simulink model "IP_LQR_Design"  (R2025b)
settings: Solver=FixedStepAuto  StartTime=0.0  StopTime=10.0  FixedStep=0.01  RelTol=1e-3
undefined symbols (not defined in the file): b, c, g, I, kb, KK, kt, l, M, m, r, Rm
libraries: vrlib x3
settings Model: Creator=jitendra  LastModifiedBy=joelalfaro
settings SolverCC: AlgebraicLoopSolver=TrustRegion
settings DataIOCC: ExternalInput=getinputstruct(op_trim1)  InitialState=getstatestruct(op_trim1)  ReturnWorkspaceOutputs=off
settings DebuggingCC: UnconnectedInputMsg=warning  UnconnectedOutputMsg=warning  UnconnectedLineMsg=warning  ArithmeticOperatorsInVariantConditions=warning
settings ModelReferenceCC: EnableRefExpFcnMdlSchedulingChecks=on
settings SFSimCC: SimUseLocalCustomCode=off  CustomCodeUndefinedFunction=UseInterfaceOnly
settings RTWCC: RTWUseLocalCustomCode=off  GPUComputeCapability=3.5

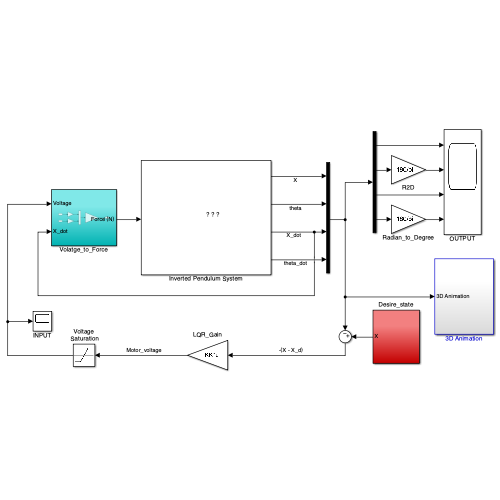
[thumbnail: Simulink's stored preview of the top-level diagram]
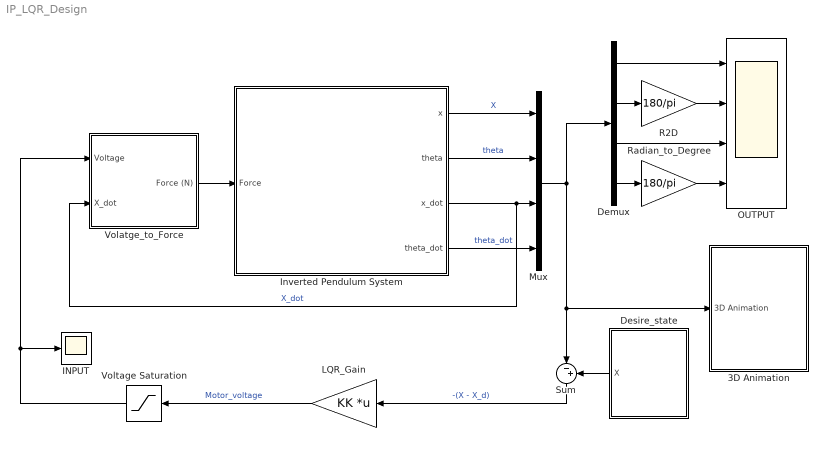
== system IP_LQR_Design ==
  3D Animation : Subsystem
  Demux : Demux
  Desire_state : Subsystem
  INPUT : Scope
      settings: ActiveDisplayYMinimum=-15  ActiveDisplayYMaximum=15
  Inverted Pendulum System : Subsystem
      mask Display: image('ip_model.png');
  LQR_Gain : Gain  Gain=KK  Multiplication=Matrix(K*u)
  Mux : Mux
  OUTPUT : Scope  NumInputPorts=4
      settings: ActiveDisplayString=4  ActiveDisplayYMinimum=-828.41149910064814  ActiveDisplayYMaximum=966.89099669448683  YLabel=\theta dot (deg/sec)
  R2D : Gain  Gain=180/pi
  Radian_to_Degree : Gain  Gain=180/pi
  Sum : Sum  Inputs=|-+
  Volatge_to_Force : Subsystem
  Voltage Saturation : Saturate  UpperLimit=12  LowerLimit=-12
  wires:
  Inverted Pendulum System/3(x_dot) -> Volatge_to_Force/2(X_dot), Mux/3  "X_dot"
  Inverted Pendulum System/2(theta) -> Mux/2  "theta"
  Inverted Pendulum System/1(x) -> Mux/1  "X"
  Inverted Pendulum System/4(theta_dot) -> Mux/4  "theta_dot"
  Mux/1 -> Demux/1, Sum/1, 3D Animation/1(3D Animation)
  LQR_Gain/1 -> Voltage Saturation/1  "Motor_voltage"
  Volatge_to_Force/1(Force (N)) -> Inverted Pendulum System/1(Force)
  Desire_state/1(X) -> Sum/2
  Sum/1 -> LQR_Gain/1  "-(X - X_d)"
  Voltage Saturation/1 -> INPUT/1, Volatge_to_Force/1(Voltage)
  Demux/2 -> R2D/1
  Demux/1 -> OUTPUT/1
  Demux/3 -> OUTPUT/3
  Demux/4 -> Radian_to_Degree/1
  R2D/1 -> OUTPUT/2
  Radian_to_Degree/1 -> OUTPUT/4

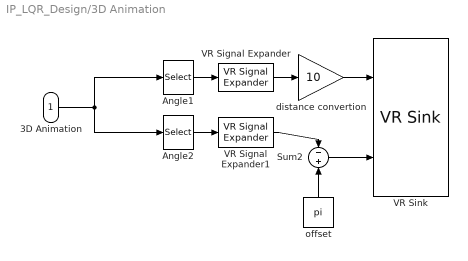
== system IP_LQR_Design/3D Animation ==
  3D Animation : Inport
  Angle1 : Selector  InputPortWidth=4  IndexOptions=Index vector (dialog)  Indices=[1]  OutputSizes=1
  Angle2 : Selector  InputPortWidth=4  IndexOptions=Index vector (dialog)  Indices=[2]  OutputSizes=1
  Sum2 : Sum  Inputs=-|+
  VR Signal Expander : vrlib/VR Signal Expander  outwidth=3  outidx=[1]
  VR Signal Expander1 : vrlib/VR Signal Expander  outwidth=4  outidx=[4]
  VR Sink : vrlib/VR Sink  InstantiateOnLoad=on  SampleTime=0.02  ViewEnable=on  RemoteChange=off  RemoteView=off  FieldsWritten=cart.translation.3.1.1.double#joint.rotation.4.1.1.double  WorldFileName=Inverted_pendulum12.wrl  AutoView=off  VideoDimensions=[]  AllowVariableSize=off  FigureProperties=[]
  distance convertion : Gain  Gain=10
  offset : Constant  Value=pi
  wires:
  VR Signal Expander/1 -> distance convertion/1
  3D Animation/1 -> Angle2/1, Angle1/1
  Angle1/1 -> VR Signal Expander/1
  Angle2/1 -> VR Signal Expander1/1
  offset/1 -> Sum2/2
  Sum2/1 -> VR Sink/2
  VR Signal Expander1/1 -> Sum2/1
  distance convertion/1 -> VR Sink/1

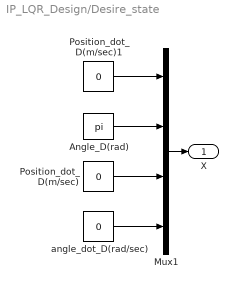
== system IP_LQR_Design/Desire_state ==
  Angle_D(rad) : Constant  Value=pi
  Mux1 : Mux
  Position_dot_D(m/sec) : Constant  Value=0
  Position_dot_D(m/sec)1 : Constant  Value=0
  angle_dot_D(rad/sec) : Constant  Value=0
  X : Outport  VectorParamsAs1DForOutWhenUnconnected=off
  wires:
  Mux1/1 -> X/1
  Position_dot_D(m/sec)/1 -> Mux1/3
  angle_dot_D(rad/sec)/1 -> Mux1/4
  Angle_D(rad)/1 -> Mux1/2
  Position_dot_D(m/sec)1/1 -> Mux1/1

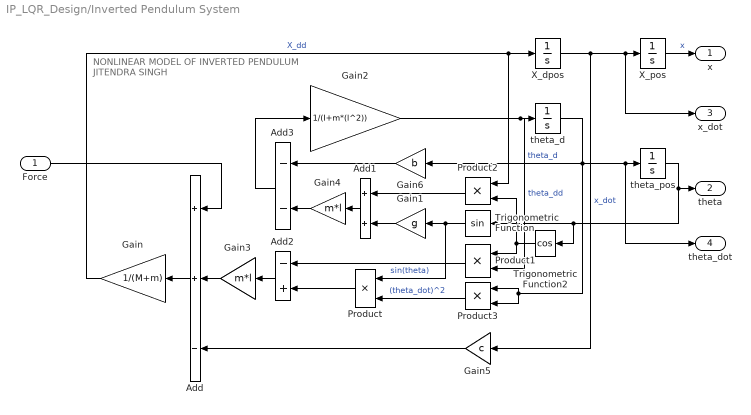
== system IP_LQR_Design/Inverted Pendulum System ==
  note: NONLINEAR MODEL OF
      | INVERTED PENDULUM
      | JITENDRA SINGH
  Force : Inport
  Add : Sum  Inputs=++-
  Add1 : Sum
  Add2 : Sum  Inputs=-+
  Add3 : Sum  Inputs=--
  Gain : Gain  Gain=1/(M+m)
  Gain1 : Gain  Gain=g
  Gain2 : Gain  Gain=1/(I+m*(l^2))
  Gain3 : Gain  Gain=m*l
  Gain4 : Gain  Gain=m*l
  Gain5 : Gain  Gain=c
  Gain6 : Gain  Gain=b
  Product{,1..3} (4 alike) : Product
  Trigonometric Function : Trigonometry
  Trigonometric Function2 : Trigonometry  Operator=cos
  X_dpos : Integrator
  X_pos : Integrator  InitialCondition=0.2
  theta_d : Integrator
  theta_pos : Integrator  InitialCondition=160*(pi/180)
  x : Outport  VectorParamsAs1DForOutWhenUnconnected=off
  theta : Outport  Port=2  VectorParamsAs1DForOutWhenUnconnected=off
  x_dot : Outport  Port=3  VectorParamsAs1DForOutWhenUnconnected=off
  theta_dot : Outport  Port=4  VectorParamsAs1DForOutWhenUnconnected=off
  wires:
  Gain5/1 -> Add/3
  Add2/1 -> Gain3/1
  Add3/1 -> Gain2/1
  Trigonometric Function2/1 -> Product2/2, Product1/1
  Trigonometric Function/1 -> Product/1, Gain1/1  "sin(theta)"
  Gain3/1 -> Add/2
  theta_d/1 -> Product3/2, Product3/1, Gain6/1, theta_dot/1, theta_pos/1  "theta_d"
  Product2/1 -> Add1/1
  Product/1 -> Add2/2
  Gain4/1 -> Add3/2
  Product3/1 -> Product/2  "(theta_dot)^2"
  X_pos/1 -> x/1  "x"
  Product1/1 -> Add2/1
  Gain/1 -> X_dpos/1, Product2/1  "X_dd"
  Add/1 -> Gain/1
  Gain2/1 -> Product1/2, theta_d/1  "theta_dd"
  Gain6/1 -> Add3/1
  theta_pos/1 -> Trigonometric Function2/1, Trigonometric Function/1, theta/1
  Force/1 -> Add/1
  Gain1/1 -> Add1/2
  X_dpos/1 -> x_dot/1, X_pos/1, Gain5/1  "x_dot"
  Add1/1 -> Gain4/1

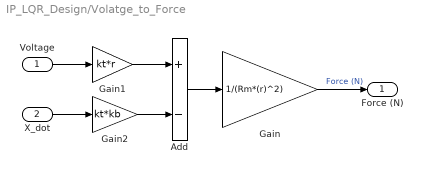
== system IP_LQR_Design/Volatge_to_Force ==
  Voltage : Inport
  X_dot : Inport  Port=2
  Add : Sum  Inputs=+-
  Gain : Gain  Gain=1/(Rm*(r)^2)
  Gain1 : Gain  Gain=kt*r
  Gain2 : Gain  Gain=kt*kb
  Force (N) : Outport  VectorParamsAs1DForOutWhenUnconnected=off
  wires:
  Gain1/1 -> Add/1
  Gain2/1 -> Add/2
  Voltage/1 -> Gain1/1
  Gain/1 -> Force (N)/1  "Force (N)"
  X_dot/1 -> Gain2/1
  Add/1 -> Gain/1
